simulink model "hrg_wa_v7_pir_study_envelope"  (R2025a)
settings: Solver=ode4  StartTime=0.0  StopTime=wl_stop  FixedStep=wl_Tc  RelTol=1e-3
PostLoadFcn:
  | addpath(fileparts(fileparts(get_param('hrg_wa_v7_pir_study_envelope','FileName')))); w7_setup(getVariable(get_param('hrg_wa_v7_pir_study_envelope','ModelWorkspace'),'v7_saved_configuration'));
model workspace (MAT data in the model file):
  v7_saved_configuration.stage = 5
  v7_saved_configuration.name = 'hrg_wa_v7_pir_study'
  v7_saved_configuration.head.sourceProfile = 'C:\Users\11725\Desktop\HRG_WA\HRG_WA_Digital_ASIC_MATLAB_v4_6_5_FRP_validation_fix\HRG_WA\config\head_default.json'
  v7_saved_configuration.head.measurementStatus = 'assumed, not a measured head'
  v7_saved_configuration.head.f0 = 5000
  v7_saved_configuration.head.Q = 2000000
  v7_saved_configuration.head.bryan = 0.277
  v7_saved_configuration.head.gamma = 0.00785398163397
  v7_saved_configuration.head.dgamma = 0.004
  v7_saved_configuration.head.dampingAxis = 0.296705972839
  v7_saved_configuration.head.splitHz = 0.08
  v7_saved_configuration.head.stiffnessAxis = 0.715584993318
  v7_saved_configuration.head.detuningHz = 0
  v7_saved_configuration.head.duffingHz = 0
  v7_saved_configuration.head.temperatureCoeff = -1.8e-05
  v7_saved_configuration.head.referenceTemperature = 25
  v7_saved_configuration.head.detect = [1  0; 0  1]
  v7_saved_configuration.head.detectPhase = [0; 0]
  v7_saved_configuration.head.drive = [1  0; 0  1]
  v7_saved_configuration.head.detectCubic = 0
  v7_saved_configuration.head.iqBits = 0
  v7_saved_configuration.head.iqFullScale = 2
  v7_saved_configuration.head.energyTarget = 1
  v7_saved_configuration.head.initialEnergy = 1
  v7_saved_configuration.head.initialTheta = 0.13962634016
  v7_saved_configuration.head.initialQuadRatio = 0
  v7_saved_configuration.head.energyKp = 4.02123859659
  v7_saved_configuration.head.energyKi = 12.6330936334
  v7_saved_configuration.head.quadKp = 6.03185789489
  v7_saved_configuration.head.quadKi = 28.4244606751
  v7_saved_configuration.head.pllKp = 1.28
  v7_saved_configuration.head.pllKi = 4.02123859659
  v7_saved_configuration.head.energyLimit = 20
  v7_saved_configuration.head.quadLimit = 2
  v7_saved_configuration.head.pllLimitHz = 2
  v7_saved_configuration.head.antiWindup = 5
  v7_saved_configuration.head.loopEnable = 1
  v7_saved_configuration.head.Ts = 0.001
  v7_saved_configuration.head.rateTau = 0.00353677651315
  v7_saved_configuration.head.energyThreshold = 0.02
  v7_saved_configuration.head.angleThreshold = 0.01
  v7_saved_configuration.head.duration = 12
  v7_saved_configuration.head.omega = 1.3962634016
  v7_saved_configuration.head.virtualRate = 0
  v7_saved_configuration.head.temperature = 25
  v7_saved_configuration.head.fullStep = 2e-06
  v7_saved_configuration.fsAdc = 40000
  v7_saved_configuration.fsPlant = 800000
  v7_saved_configuration.duration = 40
  v7_saved_configuration.seed = 20261021
  v7_saved_configuration.massKg = 1e-06
  v7_saved_configuration.displacementM = 1e-07
  v7_saved_configuration.gapM = 5e-06
  v7_saved_configuration.c0F = 1e-12
  v7_saved_configuration.cfF = 1e-12
  v7_saved_configuration.rfOhm = 1000000000
  v7_saved_configuration.biasV = 10
  v7_saved_configuration.cvBandwidthHz = 30000
  v7_saved_configuration.pgaBandwidthHz = 30000
  v7_saved_configuration.pgaGain = 1
  v7_saved_configuration.cvEnVrtHz = 1e-08
  v7_saved_configuration.cvInArtHz = 1e-14
  v7_saved_configuration.temperatureK = 298.15
  v7_saved_configuration.pgaNoiseVrtHz = 1e-08
  v7_saved_configuration.afeOffsetV = [0; 0]
  v7_saved_configuration.afeLimitV = 1.8
  v7_saved_configuration.adcBits = 0
  v7_saved_configuration.adcFsV = 2
  v7_saved_configuration.adcOffsetV = [0; 0]
  v7_saved_configuration.adcGain = [1; 1]
  v7_saved_configuration.adcInlCubic = 0
  v7_saved_configuration.jitterRmsS = 2e-09
  v7_saved_configuration.channelSkewS = 0
  v7_saved_configuration.adcDelay = 1
  v7_saved_configuration.adcArchitecture = 'nyquist'
  v7_saved_configuration.cicStages = 3
  v7_saved_configuration.fir = [0.111111111111 0.222222222222 0.333333333333 0.222222222222 0.111111111111]
  v7_saved_configuration.dacBits = 0
  v7_saved_configuration.dacFsV = 2
  v7_saved_configuration.dacDelay = 1
  v7_saved_configuration.dacInlCubic = 0
  v7_saved_configuration.dacArchitecture = 'nyquist'
  v7_saved_configuration.driveNPerV = 1e-07
  v7_saved_configuration.driverBandwidthHz = 50000
  v7_saved_configuration.driverGain = [1; 1]
  v7_saved_configuration.driverSlewVPerS = 200000
  v7_saved_configuration.driverNoiseVrtHz = 2e-08
  v7_saved_configuration.driverLimitV = 1.8
  v7_saved_configuration.feedthroughF = 0
  v7_saved_configuration.pipelineCtrl = 3
  v7_saved_configuration.iqFractionBits = 0
  v7_saved_configuration.controlFractionBits = 0
  v7_saved_configuration.antiAliasHz = 18000
  v7_saved_configuration.noiseEnable = 0
  v7_saved_configuration.circuitEnable = 1
  v7_saved_configuration.kalman = 1
  v7_saved_configuration.online = 0
  v7_saved_configuration.frp = 0
  v7_saved_configuration.calibrationPermit = 0
  v7_saved_configuration.frpSequence = 0
  v7_saved_configuration.frpFreeze = 0
  v7_saved_configuration.frpTheta = [0; 0; 0; 0; 0; 0; 0; 0; 0]
  v7_saved_configuration.matrixApply = 0
  v7_saved_configuration.compensationApply = 0
  v7_saved_configuration.temperatureCompensate = 0
  v7_saved_configuration.temperatureBiasCoefficients = [0; 0; 0]
  v7_saved_configuration.zeroRateCertified = 0
  v7_saved_configuration.virtualRate = 0
  v7_saved_configuration.inputRate = 1.3962634016
  v7_saved_configuration.inputFrequencyHz = 0
  v7_saved_configuration.inputRateAmplitude = 0
  v7_saved_configuration.temperatureC = 25
  v7_saved_configuration.temperatureRampCPerS = 0
  v7_saved_configuration.observers = 1
  v7_saved_configuration.spectra = 1
  v7_saved_configuration.maxLogPoints = 80000
  v7_saved_configuration.sdmLeak = 0.9999
  v7_saved_configuration.sdmReferenceV = 2
  v7_saved_configuration.tdmEnable = 0
  v7_saved_configuration.knownPhaseCalibrationRad = 0
  v7_saved_configuration.virtualGainCalibration = 1
  v7_saved_configuration.learnStartS = 0.25
  v7_saved_configuration.measurementStatus = 'unmeasured research assumptions; replace with measured head and interface data'
  v7_saved_configuration.scope = 'Behavioral circuit interfaces, not transistor or bit-true RTL signoff'
  v7_saved_configuration.v7.schemaVersion = 1
  v7_saved_configuration.v7.status = 'unmeasured research assumptions; replace with measured head and interface data'
  v7_saved_configuration.v7.mechanicalProfile = 'HRG_WA_Digital_ASIC_MATLAB_v4_6_5_FRP_validation_fix/HRG_WA/config/head_default.json'
  v7_saved_configuration.v7.headSimulation.Ts = 0.001
  v7_saved_configuration.v7.headSimulation.initialEnergy = 1
  v7_saved_configuration.v7.headSimulation.initialQuadRatio = 0
  v7_saved_configuration.v7.headSimulation.rateTau = 0.00353677651315
  v7_saved_configuration.v7.circuit.fsAdc = 40000
  v7_saved_configuration.v7.circuit.massKg = 1e-06
  v7_saved_configuration.v7.circuit.displacementM = 1e-07
  v7_saved_configuration.v7.circuit.gapM = 5e-06
  v7_saved_configuration.v7.circuit.c0F = 1e-12
  v7_saved_configuration.v7.circuit.biasV = 10
  v7_saved_configuration.v7.circuit.cvBandwidthHz = 30000
  v7_saved_configuration.v7.circuit.pgaBandwidthHz = 30000
  v7_saved_configuration.v7.circuit.cvEnVrtHz = 1e-08
  v7_saved_configuration.v7.circuit.cvInArtHz = 1e-14
  v7_saved_configuration.v7.circuit.temperatureK = 298.15
  v7_saved_configuration.v7.circuit.pgaNoiseVrtHz = 1e-08
  v7_saved_configuration.v7.circuit.afeOffsetV = [0; 0]
  v7_saved_configuration.v7.circuit.afeLimitV = 1.8
  v7_saved_configuration.v7.circuit.adcBits = 18
  v7_saved_configuration.v7.circuit.adcFsV = 2
  v7_saved_configuration.v7.circuit.adcOffsetV = [0; 0]
  v7_saved_configuration.v7.circuit.adcGain = [1; 1]
  v7_saved_configuration.v7.circuit.adcInlCubic = 0
  v7_saved_configuration.v7.circuit.jitterRmsS = 2e-09
  v7_saved_configuration.v7.circuit.channelSkewS = 0
  v7_saved_configuration.v7.circuit.adcDelay = 1
  v7_saved_configuration.v7.circuit.adcArchitecture = 'nyquist'
  v7_saved_configuration.v7.circuit.cicStages = 3
  v7_saved_configuration.v7.circuit.fir = [0.111111111111; 0.222222222222; 0.333333333333; 0.222222222222; 0.111111111111]
  v7_saved_configuration.v7.circuit.dacBits = 16
  v7_saved_configuration.v7.circuit.dacFsV = 2
  v7_saved_configuration.v7.circuit.dacDelay = 1
  v7_saved_configuration.v7.circuit.dacInlCubic = 0
  v7_saved_configuration.v7.circuit.dacArchitecture = 'nyquist'
  v7_saved_configuration.v7.circuit.driveNPerV = 1e-07
  v7_saved_configuration.v7.circuit.driverBandwidthHz = 50000
  v7_saved_configuration.v7.circuit.driverGain = [1; 1]
  v7_saved_configuration.v7.circuit.driverSlewVPerS = 200000
  v7_saved_configuration.v7.circuit.driverNoiseVrtHz = 2e-08
  v7_saved_configuration.v7.circuit.driverLimitV = 1.8
  v7_saved_configuration.v7.circuit.feedthroughF = 0
  v7_saved_configuration.v7.circuit.pipelineCtrl = 3
  v7_saved_configuration.v7.circuit.iqFractionBits = 22
  v7_saved_configuration.v7.circuit.controlFractionBits = 22
  v7_saved_configuration.v7.circuit.antiAliasHz = 18000
  v7_saved_configuration.v7.fsPlant = 800000
  v7_saved_configuration.v7.duration = 2
  v7_saved_configuration.v7.readoutMode = 'charge'
  v7_saved_configuration.v7.charge.rfOhm = 1000000000
  v7_saved_configuration.v7.charge.cfF = 1e-12
  v7_saved_configuration.v7.charge.pgaGain = 1
  v7_saved_configuration.v7.tia.rfOhm = 1000000
  v7_saved_configuration.v7.tia.cfF = 1e-12
  v7_saved_configuration.v7.tia.pgaGain = 31.8309886184
  v7_saved_configuration.v7.loopNaturalHz = [0.8; 1.2; 0.8]
  v7_saved_configuration.v7.dampingRatio = 0.8
  v7_saved_configuration.v7.controlMode = 'PIR'
  v7_saved_configuration.v7.resonantGain = [0.4; 1.2; 0]
  v7_saved_configuration.v7.resonantLeakRadS = 0.04
  v7_saved_configuration.v7.resonantMinimumRadS = 0.15
  v7_saved_configuration.v7.resonantMaximumRadS = 25
  v7_saved_configuration.v7.frequencyEstimateTauS = 0.1
  v7_saved_configuration.v7.slewPerS = [500; 100; 100]
  v7_saved_configuration.v7.startupEnable = 0
  v7_saved_configuration.v7.startupAmplitudePerS = 4
  v7_saved_configuration.v7.startupSwitchEnergy = 0.25
  v7_saved_configuration.v7.startupTimeoutS = 1.5
  v7_saved_configuration.v7.startupDirectionRad = 0
  v7_saved_configuration.v7.tdmMode = 'continuous'
  v7_saved_configuration.v7.slotCycles = [1; 1; 2; 1]
  v7_saved_configuration.v7.readBlankCycles = 0.25
  v7_saved_configuration.v7.acquisitionTauS = 2e-06
  v7_saved_configuration.v7.unloadTauS = 2e-06
  v7_saved_configuration.v7.sampleCapF = 1e-11
  v7_saved_configuration.v7.switchChargeC = [0; 0]
  v7_saved_configuration.v7.actuationMode = 'linear'
  v7_saved_configuration.v7.driveBiasV = 10
  v7_saved_configuration.v7.electrostaticForceScale = 0.025
  v7_saved_configuration.v7.budget.angleRmsRad = 1e-06
  v7_saved_configuration.v7.budget.noiseBandwidthHz = 100
  v7_saved_configuration.v7.budget.startupTimeS = 0.1
  v7_saved_configuration.v7.profile = 'C:\Users\11725\Desktop\HRG_WA\HRG_WA_simulink\literature_v7\profile.json'
  v7_saved_configuration.v7.senseCalibration = 0.228707119333+1.04243935371i
  v7_saved_configuration.v7.driveCalibration = 0.297893136802+0.987329357138i
  v7_saved_configuration.v7.nominalGram = [0.5  0; 0  0.5]
  v7_saved_configuration.cvEquivalentNoiseVrtHz = 3.43925280635e-07
undefined symbols (not defined in the file): w7_control_tick, w7_iq, wa_plant_rhs, wl_c, wl_env_drive, wl_env_sense, wl_env_z0, wl_fir, wl_input, wl_invariants, wl_p, wl_Tc
settings Model: Creator=11725  LastModifiedBy=11725
settings DataIOCC: SaveOutput=off
settings DebuggingCC: AlgebraicLoopMsg=error

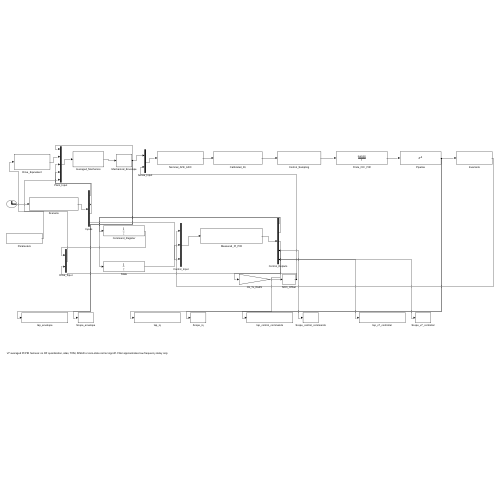
[thumbnail: Simulink's stored preview of the top-level diagram]
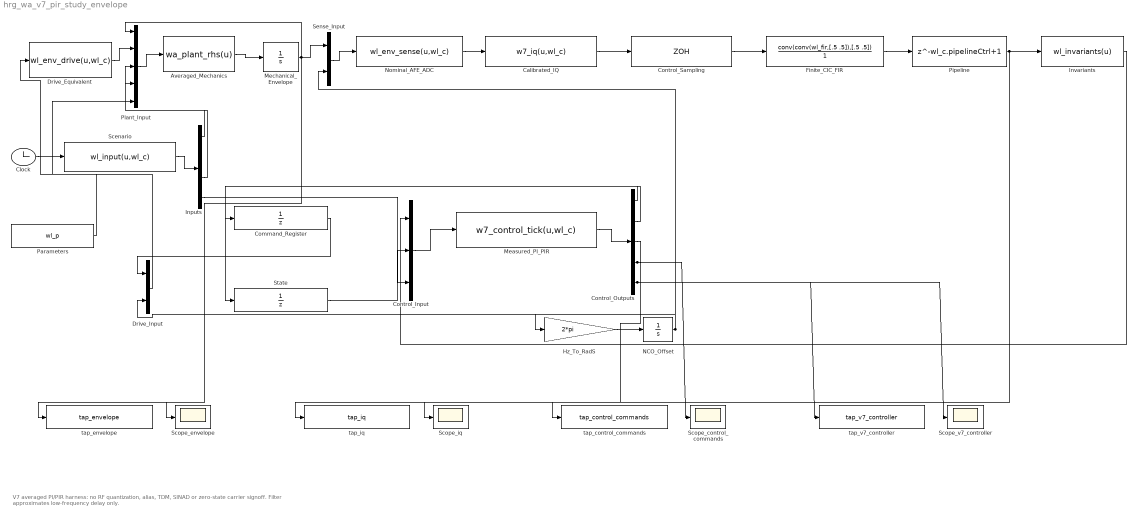
== system hrg_wa_v7_pir_study_envelope ==
  note: V7 averaged PI/PIR harness: no RF quantization, alias, TDM, SINAD or zero-state carrier signoff. Filter approximates low-frequency delay only.
  Averaged_Mechanics : MATLABFcn  MATLABFcn=wa_plant_rhs(u)  OutputDimensions=4
  Calibrated_IQ : MATLABFcn  MATLABFcn=w7_iq(u,wl_c)  OutputDimensions=4
  Clock : Clock
  Command_Register : UnitDelay  InitialCondition=zeros(4,1)  SampleTime=wl_Tc  HasFrameUpgradeWarning=on
  Control_Input : Mux  Inputs=3
  Control_Outputs : Demux  Outputs=[17 4 1 3 8]
  Control_Sampling : ZeroOrderHold  SampleTime=wl_Tc
  Drive_Equivalent : MATLABFcn  MATLABFcn=wl_env_drive(u,wl_c)  OutputDimensions=4
  Drive_Input : Mux  Inputs=2
  Finite_CIC_FIR : DiscreteFilter  Numerator=conv(conv(wl_fir,[.5 .5]),[.5 .5])  Denominator=1  SampleTime=wl_Tc
  Hz_To_RadS : Gain  Gain=2*pi
  Inputs : Demux  Outputs=[1 1 1 1]
  Invariants : MATLABFcn  MATLABFcn=wl_invariants(u)  OutputDimensions=10
  Measured_PI_PIR : MATLABFcn  MATLABFcn=w7_control_tick(u,wl_c)  OutputDimensions=33
  Mechanical_Envelope : Integrator  InitialCondition=wl_env_z0
  NCO_Offset : Integrator
  Nominal_AFE_ADC : MATLABFcn  MATLABFcn=wl_env_sense(u,wl_c)  OutputDimensions=4
  Parameters : Constant  Value=wl_p
  Pipeline : Delay  DelayLength=wl_c.pipelineCtrl+1  InitialCondition=0  SampleTime=wl_Tc
  Plant_Input : Mux  Inputs=5
  Scenario : MATLABFcn  MATLABFcn=wl_input(u,wl_c)  OutputDimensions=4
  Scope_control_commands : Scope
  Scope_envelope : Scope
  Scope_iq : Scope
  Scope_v7_controller : Scope
  Sense_Input : Mux  Inputs=2
  State : UnitDelay  InitialCondition=zeros(17,1)  SampleTime=wl_Tc  HasFrameUpgradeWarning=on
  tap_control_commands : ToWorkspace  VariableName=tap_control_commands  SaveFormat=Timeseries  SampleTime=-1
  tap_envelope : ToWorkspace  VariableName=tap_envelope  SaveFormat=Timeseries  SampleTime=-1
  tap_iq : ToWorkspace  VariableName=tap_iq  SaveFormat=Timeseries  SampleTime=-1
  tap_v7_controller : ToWorkspace  VariableName=tap_v7_controller  SaveFormat=Timeseries  SampleTime=-1
  wires:
  Clock/1 -> Scenario/1
  Scenario/1 -> Inputs/1
  Mechanical_Envelope/1 -> Plant_Input/1, Sense_Input/1, tap_envelope/1, Scope_envelope/1
  Inputs/1 -> Plant_Input/3
  Inputs/3 -> Plant_Input/4
  Parameters/1 -> Plant_Input/5
  Plant_Input/1 -> Averaged_Mechanics/1
  Averaged_Mechanics/1 -> Mechanical_Envelope/1
  NCO_Offset/1 -> Sense_Input/2, Drive_Input/2
  Sense_Input/1 -> Nominal_AFE_ADC/1
  Nominal_AFE_ADC/1 -> Calibrated_IQ/1
  Calibrated_IQ/1 -> Control_Sampling/1
  Control_Sampling/1 -> Finite_CIC_FIR/1
  Finite_CIC_FIR/1 -> Pipeline/1
  Pipeline/1 -> Invariants/1, tap_iq/1, Scope_iq/1
  Invariants/1 -> Control_Input/1
  Inputs/4 -> Control_Input/3
  State/1 -> Control_Input/2
  Control_Input/1 -> Measured_PI_PIR/1
  Measured_PI_PIR/1 -> Control_Outputs/1
  Control_Outputs/1 -> State/1
  Control_Outputs/3 -> Hz_To_RadS/1
  Hz_To_RadS/1 -> NCO_Offset/1
  Control_Outputs/2 -> Command_Register/1
  Command_Register/1 -> Drive_Input/1
  Drive_Input/1 -> Drive_Equivalent/1
  Drive_Equivalent/1 -> Plant_Input/2
  Control_Outputs/4 -> tap_control_commands/1, Scope_control_commands/1
  Control_Outputs/5 -> tap_v7_controller/1, Scope_v7_controller/1
